simulink model "V9_Whitebox_Resource_Network"  (R2026a)
settings: Solver=FixedStepDiscrete  StartTime=0  StopTime=2159  FixedStep=1
undefined symbols (not defined in the file or in its folder): v9_coal_conversion, v9_controller, v9_eta_charge, v9_eta_discharge, v9_gas_conversion, v9_initial_fuel, v9_initial_soc, v9_initial_thermal, v9_trace
settings Model: Creator=Y9000P  LastModifiedBy=Y9000P

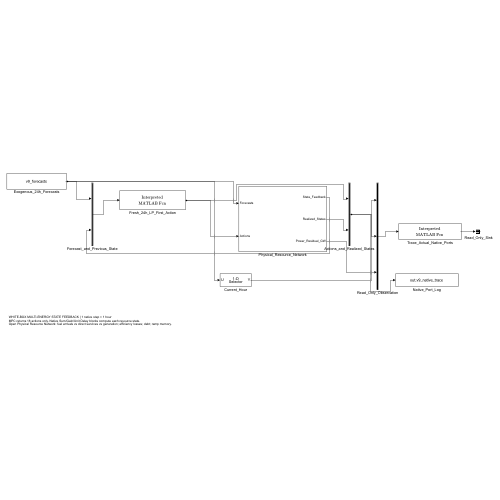
[thumbnail: Simulink's stored preview of the top-level diagram]
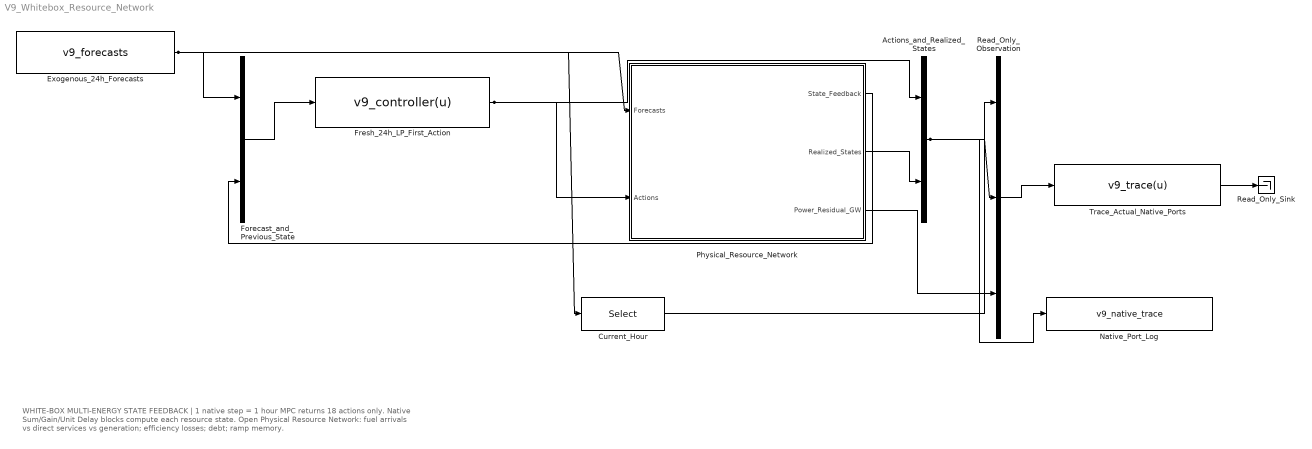
== system V9_Whitebox_Resource_Network ==
  note: WHITE-BOX MULTI-ENERGY STATE FEEDBACK | 1 native step = 1 hour
      | MPC returns 18 actions only. Native Sum/Gain/Unit Delay blocks compute each resource state.
      | Open Physical Resource Network: fuel arrivals vs direct services vs generation; efficiency losses; debt; ramp memory.
  Actions_and_Realized_States : Mux  Inputs=2
  Current_Hour : Selector  InputPortWidth=337  IndexOptions=Index vector (dialog)  Indices=1  OutputSizes=1
  Exogenous_24h_Forecasts : FromWorkspace  VariableName=v9_forecasts  Interpolate=off  OutputAfterFinalValue=Holding final value
  Forecast_and_Previous_State : Mux  Inputs=2
  Fresh_24h_LP_First_Action : MATLABFcn  MATLABFcn=v9_controller(u)  OutputDimensions=18
  Native_Port_Log : ToWorkspace  VariableName=v9_native_trace  SampleTime=-1
  Physical_Resource_Network : Subsystem
  Read_Only_Observation : Mux  Inputs=3
  Read_Only_Sink : Terminator
  Trace_Actual_Native_Ports : MATLABFcn  MATLABFcn=v9_trace(u)  OutputDimensions=1
  wires:
  Exogenous_24h_Forecasts/1 -> Forecast_and_Previous_State/1, Physical_Resource_Network/1(Forecasts), Current_Hour/1
  Physical_Resource_Network/1(State_Feedback) -> Forecast_and_Previous_State/2
  Forecast_and_Previous_State/1 -> Fresh_24h_LP_First_Action/1
  Fresh_24h_LP_First_Action/1 -> Physical_Resource_Network/2(Actions), Actions_and_Realized_States/1
  Physical_Resource_Network/2(Realized_States) -> Actions_and_Realized_States/2
  Current_Hour/1 -> Read_Only_Observation/1
  Actions_and_Realized_States/1 -> Read_Only_Observation/2, Native_Port_Log/1
  Physical_Resource_Network/3(Power_Residual_GW) -> Read_Only_Observation/3
  Read_Only_Observation/1 -> Trace_Actual_Native_Ports/1
  Trace_Actual_Native_Ports/1 -> Read_Only_Sink/1

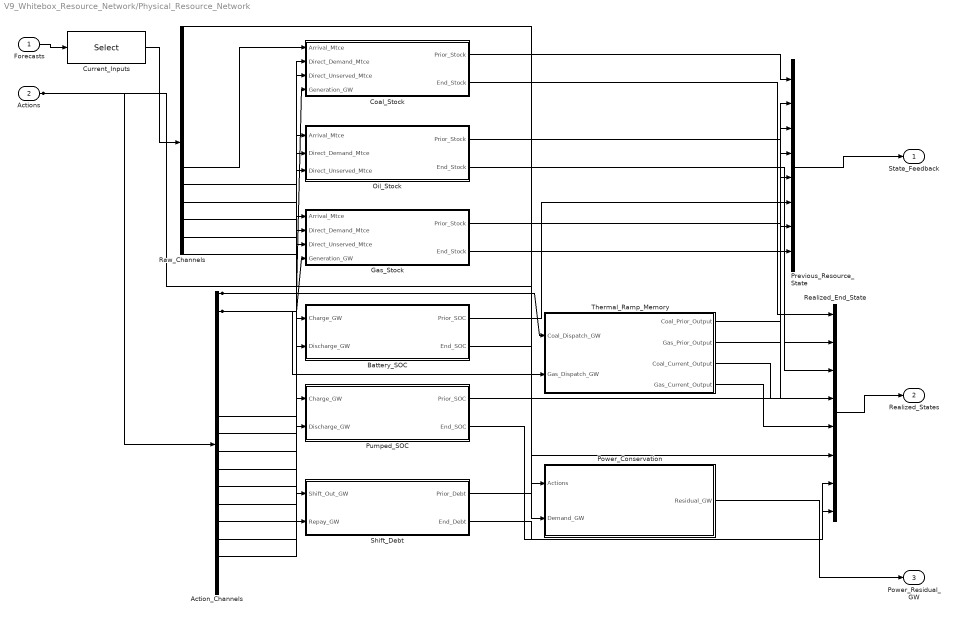
== system V9_Whitebox_Resource_Network/Physical_Resource_Network ==
  Forecasts : Inport
  Actions : Inport  Port=2
  Action_Channels : Demux  Outputs=18
  Battery_SOC : Subsystem
  Coal_Stock : Subsystem
  Current_Inputs : Selector  InputPortWidth=337  IndexOptions=Index vector (dialog)  Indices=[2:15]  OutputSizes=1
  Gas_Stock : Subsystem
  Oil_Stock : Subsystem
  Power_Conservation : Subsystem
  Previous_Resource_State : Mux  Inputs=8
  Pumped_SOC : Subsystem
  Raw_Channels : Demux  Outputs=14
  Realized_End_State : Mux  Inputs=8
  Shift_Debt : Subsystem
  Thermal_Ramp_Memory : Subsystem
  State_Feedback : Outport
  Realized_States : Outport  Port=2
  Power_Residual_GW : Outport  Port=3
  wires:
  Forecasts/1 -> Current_Inputs/1
  Current_Inputs/1 -> Raw_Channels/1
  Actions/1 -> Action_Channels/1, Power_Conservation/1(Actions)
  Raw_Channels/9 -> Coal_Stock/1(Arrival_Mtce)
  Raw_Channels/12 -> Coal_Stock/2(Direct_Demand_Mtce)
  Action_Channels/12 -> Coal_Stock/3(Direct_Unserved_Mtce)
  Action_Channels/1 -> Coal_Stock/4(Generation_GW), Thermal_Ramp_Memory/1(Coal_Dispatch_GW)
  Raw_Channels/10 -> Oil_Stock/1(Arrival_Mtce)
  Raw_Channels/13 -> Oil_Stock/2(Direct_Demand_Mtce)
  Action_Channels/13 -> Oil_Stock/3(Direct_Unserved_Mtce)
  Raw_Channels/11 -> Gas_Stock/1(Arrival_Mtce)
  Raw_Channels/14 -> Gas_Stock/2(Direct_Demand_Mtce)
  Action_Channels/14 -> Gas_Stock/3(Direct_Unserved_Mtce)
  Action_Channels/2 -> Gas_Stock/4(Generation_GW), Thermal_Ramp_Memory/2(Gas_Dispatch_GW)
  Action_Channels/8 -> Battery_SOC/1(Charge_GW)
  Action_Channels/9 -> Battery_SOC/2(Discharge_GW)
  Action_Channels/10 -> Pumped_SOC/1(Charge_GW)
  Action_Channels/11 -> Pumped_SOC/2(Discharge_GW)
  Action_Channels/15 -> Shift_Debt/1(Shift_Out_GW)
  Action_Channels/16 -> Shift_Debt/2(Repay_GW)
  Raw_Channels/1 -> Power_Conservation/2(Demand_GW)
  Coal_Stock/1(Prior_Stock) -> Previous_Resource_State/1
  Coal_Stock/2(End_Stock) -> Realized_End_State/1
  Oil_Stock/1(Prior_Stock) -> Previous_Resource_State/2
  Oil_Stock/2(End_Stock) -> Realized_End_State/2
  Gas_Stock/1(Prior_Stock) -> Previous_Resource_State/3
  Gas_Stock/2(End_Stock) -> Realized_End_State/3
  Thermal_Ramp_Memory/1(Coal_Prior_Output) -> Previous_Resource_State/4
  Thermal_Ramp_Memory/3(Coal_Current_Output) -> Realized_End_State/4
  Thermal_Ramp_Memory/2(Gas_Prior_Output) -> Previous_Resource_State/5
  Thermal_Ramp_Memory/4(Gas_Current_Output) -> Realized_End_State/5
  Battery_SOC/1(Prior_SOC) -> Previous_Resource_State/6
  Battery_SOC/2(End_SOC) -> Realized_End_State/6
  Pumped_SOC/1(Prior_SOC) -> Previous_Resource_State/7
  Pumped_SOC/2(End_SOC) -> Realized_End_State/7
  Shift_Debt/1(Prior_Debt) -> Previous_Resource_State/8
  Shift_Debt/2(End_Debt) -> Realized_End_State/8
  Previous_Resource_State/1 -> State_Feedback/1
  Realized_End_State/1 -> Realized_States/1
  Power_Conservation/1(Residual_GW) -> Power_Residual_GW/1

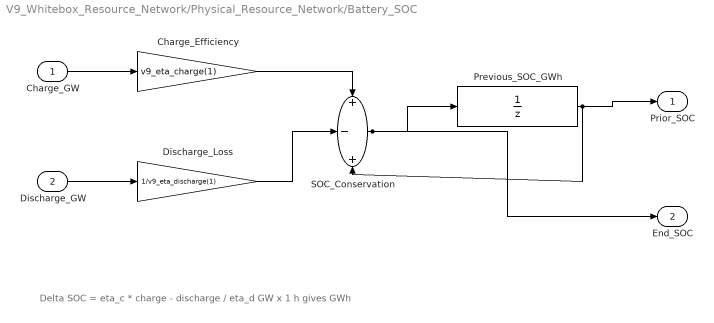
== system V9_Whitebox_Resource_Network/Physical_Resource_Network/Battery_SOC ==
  note: Delta SOC = eta_c * charge - discharge / eta_d
      | GW x 1 h gives GWh
  Charge_GW : Inport
  Discharge_GW : Inport  Port=2
  Charge_Efficiency : Gain  Gain=v9_eta_charge(1)
  Discharge_Loss : Gain  Gain=1/v9_eta_discharge(1)
  Previous_SOC_GWh : UnitDelay  InitialCondition=v9_initial_soc(1)
  SOC_Conservation : Sum  Inputs=+-+
  Prior_SOC : Outport
  End_SOC : Outport  Port=2
  wires:
  Charge_GW/1 -> Charge_Efficiency/1
  Discharge_GW/1 -> Discharge_Loss/1
  Charge_Efficiency/1 -> SOC_Conservation/1
  Discharge_Loss/1 -> SOC_Conservation/2
  Previous_SOC_GWh/1 -> SOC_Conservation/3, Prior_SOC/1
  SOC_Conservation/1 -> Previous_SOC_GWh/1, End_SOC/1

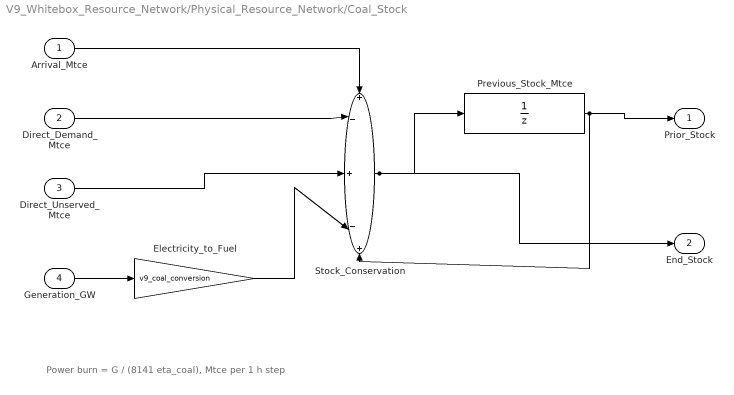
== system V9_Whitebox_Resource_Network/Physical_Resource_Network/Coal_Stock ==
  note: Power burn = G / (8141 eta_coal), Mtce per 1 h step
  Arrival_Mtce : Inport
  Direct_Demand_Mtce : Inport  Port=2
  Direct_Unserved_Mtce : Inport  Port=3
  Generation_GW : Inport  Port=4
  Electricity_to_Fuel : Gain  Gain=v9_coal_conversion
  Previous_Stock_Mtce : UnitDelay  InitialCondition=v9_initial_fuel(1)
  Stock_Conservation : Sum  Inputs=+-+-+
  Prior_Stock : Outport
  End_Stock : Outport  Port=2
  wires:
  Generation_GW/1 -> Electricity_to_Fuel/1
  Arrival_Mtce/1 -> Stock_Conservation/1
  Direct_Demand_Mtce/1 -> Stock_Conservation/2
  Direct_Unserved_Mtce/1 -> Stock_Conservation/3
  Electricity_to_Fuel/1 -> Stock_Conservation/4
  Previous_Stock_Mtce/1 -> Stock_Conservation/5, Prior_Stock/1
  Stock_Conservation/1 -> Previous_Stock_Mtce/1, End_Stock/1

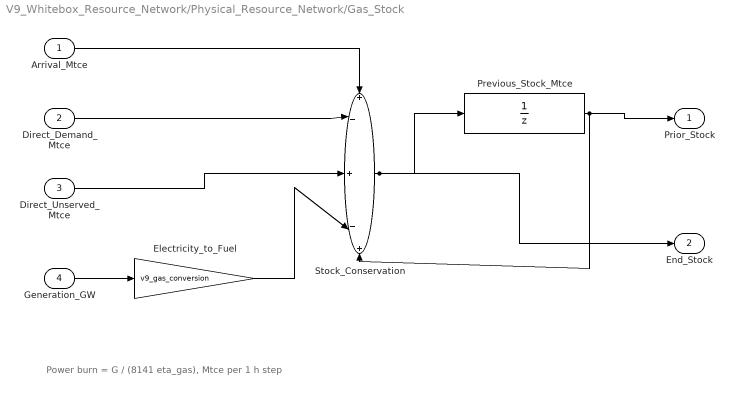
== system V9_Whitebox_Resource_Network/Physical_Resource_Network/Gas_Stock ==
  note: Power burn = G / (8141 eta_gas), Mtce per 1 h step
  Arrival_Mtce : Inport
  Direct_Demand_Mtce : Inport  Port=2
  Direct_Unserved_Mtce : Inport  Port=3
  Generation_GW : Inport  Port=4
  Electricity_to_Fuel : Gain  Gain=v9_gas_conversion
  Previous_Stock_Mtce : UnitDelay  InitialCondition=v9_initial_fuel(3)
  Stock_Conservation : Sum  Inputs=+-+-+
  Prior_Stock : Outport
  End_Stock : Outport  Port=2
  wires:
  Generation_GW/1 -> Electricity_to_Fuel/1
  Arrival_Mtce/1 -> Stock_Conservation/1
  Direct_Demand_Mtce/1 -> Stock_Conservation/2
  Direct_Unserved_Mtce/1 -> Stock_Conservation/3
  Electricity_to_Fuel/1 -> Stock_Conservation/4
  Previous_Stock_Mtce/1 -> Stock_Conservation/5, Prior_Stock/1
  Stock_Conservation/1 -> Previous_Stock_Mtce/1, End_Stock/1

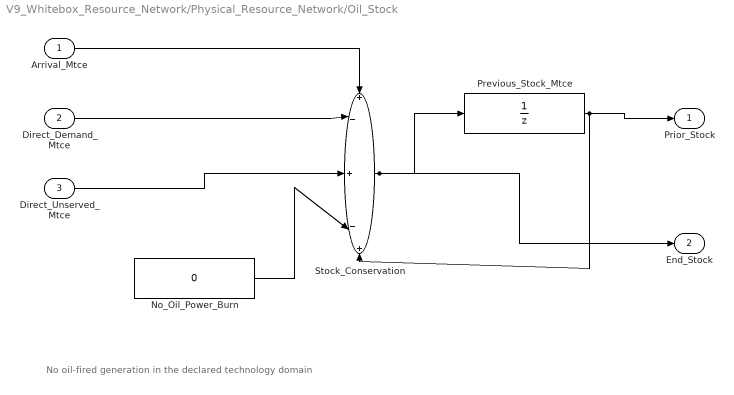
== system V9_Whitebox_Resource_Network/Physical_Resource_Network/Oil_Stock ==
  note: No oil-fired generation in the declared technology domain
  Arrival_Mtce : Inport
  Direct_Demand_Mtce : Inport  Port=2
  Direct_Unserved_Mtce : Inport  Port=3
  No_Oil_Power_Burn : Constant  Value=0
  Previous_Stock_Mtce : UnitDelay  InitialCondition=v9_initial_fuel(2)
  Stock_Conservation : Sum  Inputs=+-+-+
  Prior_Stock : Outport
  End_Stock : Outport  Port=2
  wires:
  Arrival_Mtce/1 -> Stock_Conservation/1
  Direct_Demand_Mtce/1 -> Stock_Conservation/2
  Direct_Unserved_Mtce/1 -> Stock_Conservation/3
  No_Oil_Power_Burn/1 -> Stock_Conservation/4
  Previous_Stock_Mtce/1 -> Stock_Conservation/5, Prior_Stock/1
  Stock_Conservation/1 -> Previous_Stock_Mtce/1, End_Stock/1

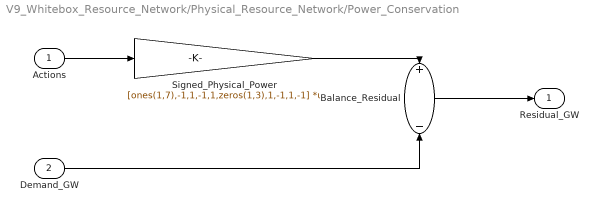
== system V9_Whitebox_Resource_Network/Physical_Resource_Network/Power_Conservation ==
  Actions : Inport
  Demand_GW : Inport  Port=2
  Balance_Residual : Sum  Inputs=+-
  Signed_Physical_Power : Gain  Gain=[ones(1,7),-1,1,-1,1,zeros(1,3),1,-1,1,-1]  Multiplication=Matrix(K*u)
  Residual_GW : Outport
  wires:
  Actions/1 -> Signed_Physical_Power/1
  Signed_Physical_Power/1 -> Balance_Residual/1
  Demand_GW/1 -> Balance_Residual/2
  Balance_Residual/1 -> Residual_GW/1

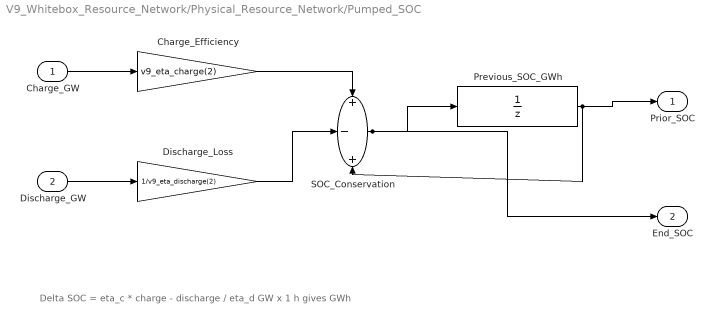
== system V9_Whitebox_Resource_Network/Physical_Resource_Network/Pumped_SOC ==
  note: Delta SOC = eta_c * charge - discharge / eta_d
      | GW x 1 h gives GWh
  Charge_GW : Inport
  Discharge_GW : Inport  Port=2
  Charge_Efficiency : Gain  Gain=v9_eta_charge(2)
  Discharge_Loss : Gain  Gain=1/v9_eta_discharge(2)
  Previous_SOC_GWh : UnitDelay  InitialCondition=v9_initial_soc(2)
  SOC_Conservation : Sum  Inputs=+-+
  Prior_SOC : Outport
  End_SOC : Outport  Port=2
  wires:
  Charge_GW/1 -> Charge_Efficiency/1
  Discharge_GW/1 -> Discharge_Loss/1
  Charge_Efficiency/1 -> SOC_Conservation/1
  Discharge_Loss/1 -> SOC_Conservation/2
  Previous_SOC_GWh/1 -> SOC_Conservation/3, Prior_SOC/1
  SOC_Conservation/1 -> Previous_SOC_GWh/1, End_SOC/1

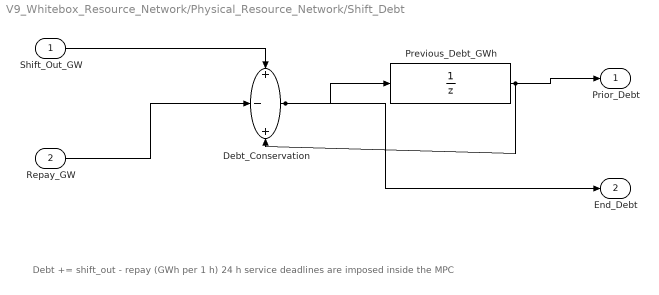
== system V9_Whitebox_Resource_Network/Physical_Resource_Network/Shift_Debt ==
  note: Debt += shift_out - repay (GWh per 1 h)
      | 24 h service deadlines are imposed inside the MPC
  Shift_Out_GW : Inport
  Repay_GW : Inport  Port=2
  Debt_Conservation : Sum  Inputs=+-+
  Previous_Debt_GWh : UnitDelay
  Prior_Debt : Outport
  End_Debt : Outport  Port=2
  wires:
  Shift_Out_GW/1 -> Debt_Conservation/1
  Repay_GW/1 -> Debt_Conservation/2
  Previous_Debt_GWh/1 -> Debt_Conservation/3, Prior_Debt/1
  Debt_Conservation/1 -> Previous_Debt_GWh/1, End_Debt/1

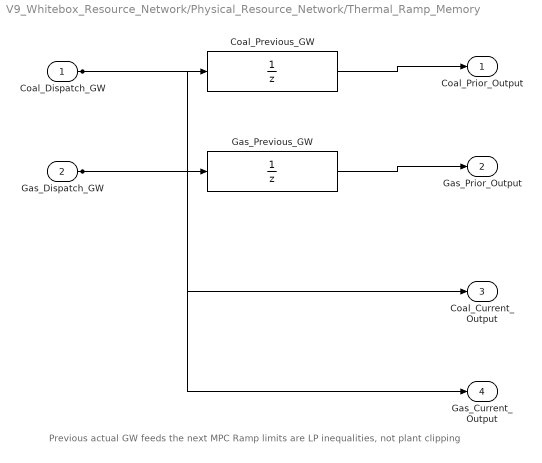
== system V9_Whitebox_Resource_Network/Physical_Resource_Network/Thermal_Ramp_Memory ==
  note: Previous actual GW feeds the next MPC
      | Ramp limits are LP inequalities, not plant clipping
  Coal_Dispatch_GW : Inport
  Gas_Dispatch_GW : Inport  Port=2
  Coal_Previous_GW : UnitDelay  InitialCondition=v9_initial_thermal(1)
  Gas_Previous_GW : UnitDelay  InitialCondition=v9_initial_thermal(2)
  Coal_Prior_Output : Outport
  Gas_Prior_Output : Outport  Port=2
  Coal_Current_Output : Outport  Port=3
  Gas_Current_Output : Outport  Port=4
  wires:
  Coal_Dispatch_GW/1 -> Coal_Previous_GW/1, Coal_Current_Output/1
  Coal_Previous_GW/1 -> Coal_Prior_Output/1
  Gas_Dispatch_GW/1 -> Gas_Previous_GW/1, Gas_Current_Output/1
  Gas_Previous_GW/1 -> Gas_Prior_Output/1
